simulink model "hovercraft_cascade_control"  (R2024a)
settings: Solver=VariableStepAuto  StartTime=0.0  StopTime=150  RelTol=1e-3
libraries: mpclib x1
settings Model: Creator=ettor  LastModifiedBy=ettor
settings SolverCC: MaxConsecutiveMinStep=100

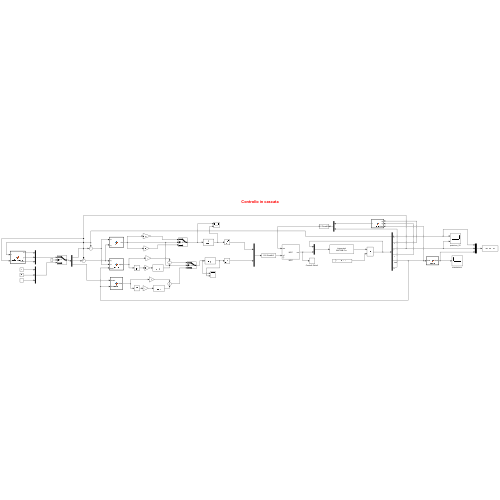
[thumbnail: Simulink's stored preview of the top-level diagram]
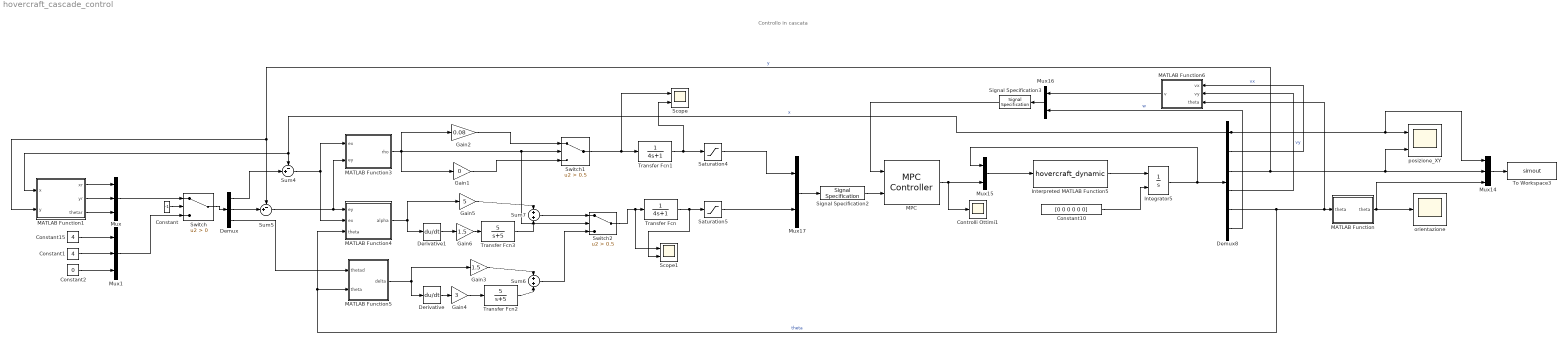
== system hovercraft_cascade_control ==
  note: Controllo in cascata
  Constant : Constant  Value=-1
  Constant1 : Constant  Value=4
  Constant10 : Constant  Value=[0 0 0 0 0 0]
  Constant15 : Constant  Value=4
  Constant2 : Constant  Value=0
  Controlli Ottimi1 : Scope
  Demux : Demux  Outputs=3
  Demux8 : Demux  Outputs=6
  Derivative : Derivative
  Derivative1 : Derivative
  Gain1 : Gain  Gain=0
  Gain2 : Gain  Gain=0.08
  Gain3 : Gain  Gain=1.5
  Gain4 : Gain  Gain=3
  Gain5 : Gain  Gain=5
  Gain6 : Gain  Gain=1.5
  Integrator5 : Integrator  InitialConditionSource=external
  Interpreted MATLAB Function5 : MATLABFcn  MATLABFcn=hovercraft_dynamic
  MATLAB Function : MATLAB Function  TreatAsAtomicUnit=on
  MATLAB Function1 : MATLAB Function  TreatAsAtomicUnit=on
  MATLAB Function3 : MATLAB Function  TreatAsAtomicUnit=on
  MATLAB Function4 : MATLAB Function  TreatAsAtomicUnit=on
  MATLAB Function5 : MATLAB Function  TreatAsAtomicUnit=on
  MATLAB Function6 : MATLAB Function  TreatAsAtomicUnit=on
  MPC : mpclib/MPC Controller  SCDEnableBlockLinearizationSpecification=on  mpcobj=mpc_simp  is_multiple=0  enable_value=0  return_u0=off  updateMPCinCallerWorkspace=on  md_inport=off  mv_inport=off  uref_inport=off  return_cost=off  return_mvseq=off  return_qpstatus=off  return_xseq=off  return_state=off  return_ovseq=off  state_inport=off  umin_inport=off  umax_inport=off  ymin_inport=off  ymax_inport=off  cc_inport=off  ywt_inport=off  uwt_inport=off  duwt_inport=off  rhoeps_inport=off  pm_inport=off  MaximumP=10  HorizonChoice=FixedHorizon  n_ts=0.05  n_p=80  n_mv=2  n_md=0  n_ud=0  n_mo=2  n_uo=0  BlockDataType=double  SampleTimeInherited=off  switch_inport=off
  Mux : Mux  Inputs=3
  Mux1 : Mux  Inputs=3
  Mux14 : Mux  Inputs=3
  Mux15 : Mux  Inputs=2
  Mux16 : Mux  Inputs=2
  Mux17 : Mux  Inputs=2
  Saturation4 : Saturate  UpperLimit=12  LowerLimit=-6
  Saturation5 : Saturate  UpperLimit=0.9  LowerLimit=-0.9
  Scope : Scope  NumInputPorts=2
  Scope1 : Scope  NumInputPorts=2
  Signal Specification2 : SignalSpecification  Dimensions=2
  Signal Specification3 : SignalSpecification  Dimensions=2
  Sum4 : Sum  Inputs=-+|
  Sum5 : Sum  Inputs=-+|
  Sum6 : Sum  Inputs=+|+
  Sum7 : Sum  Inputs=+|+
  Switch : Switch  Criteria=u2 > Threshold  SaturateOnIntegerOverflow=off  InputSameDT=off
  Switch1 : Switch  Criteria=u2 > Threshold  Threshold=0.5  SaturateOnIntegerOverflow=off  InputSameDT=off
  Switch2 : Switch  Criteria=u2 > Threshold  Threshold=0.5  SaturateOnIntegerOverflow=off  InputSameDT=off
  To Workspace3 : ToWorkspace  VariableName=simout  SaveFormat=Structure With Time  SampleTime=-1
      settings: Save2DSignal=2-D array (concatenate along first dimension)
  Transfer Fcn : TransferFcn  Denominator=[4 1]
  Transfer Fcn1 : TransferFcn  Denominator=[4 1]
  Transfer Fcn2 : TransferFcn  Numerator=5  Denominator=[1 5]
  Transfer Fcn3 : TransferFcn  Numerator=[5]  Denominator=[1 5]
  "orientazione " : Scope
  posizione_XY : Scope  NumInputPorts=2
  wires:
  Gain4/1 -> Transfer Fcn2/1
  Gain6/1 -> Transfer Fcn3/1
  Derivative1/1 -> Gain6/1
  Transfer Fcn2/1 -> Sum6/2
  Gain5/1 -> Sum7/1
  Demux8/5 -> MATLAB Function/1("theta "), MATLAB Function6/3(theta), MATLAB Function5/2(theta), MATLAB Function4/3(theta)  "theta"
  Mux15/1 -> Interpreted MATLAB Function5/1
  MPC/1 -> Controlli Ottimi1/1, Mux15/2
  Saturation5/1 -> Mux17/2
  Integrator5/1 -> Mux15/1, Demux8/1
  Demux8/6 -> Mux16/2  "w"
  Mux16/1 -> Signal Specification3/1
  Interpreted MATLAB Function5/1 -> Integrator5/1
  Saturation4/1 -> Mux17/1
  Transfer Fcn/1 -> Scope1/2, Saturation5/1
  Constant10/1 -> Integrator5/2
  Demux8/4 -> MATLAB Function6/2(vy)  "vy"
  Mux14/1 -> To Workspace3/1
  Demux8/3 -> posizione_XY/2, Mux14/2, Sum5/1, MATLAB Function1/2(y)  "y"
  Demux8/2 -> MATLAB Function6/1(vx)  "vx"
  MATLAB Function5/1(delta) -> Gain3/1, Derivative/1
  Mux17/1 -> Signal Specification2/1
  Gain3/1 -> Sum6/1
  Transfer Fcn1/1 -> Scope/2, Saturation4/1
  Demux8/1 -> Mux14/1, posizione_XY/1, MATLAB Function1/1(x), Sum4/1  "x"
  Transfer Fcn3/1 -> Sum7/2
  Signal Specification2/1 -> MPC/2
  Derivative/1 -> Gain4/1
  Switch2/1 -> Scope1/1, Transfer Fcn/1
  Sum7/1 -> Switch2/1
  MATLAB Function3/1(rho) -> Gain2/1, Switch2/2, Switch1/2, Gain1/1
  MATLAB Function4/1(alpha) -> Gain5/1, Derivative1/1
  Gain2/1 -> Switch1/1
  Switch1/1 -> Scope/1, Transfer Fcn1/1
  Sum6/1 -> Switch2/3
  Gain1/1 -> Switch1/3
  Sum4/1 -> MATLAB Function4/2(ex), MATLAB Function3/1(ex)
  Sum5/1 -> MATLAB Function4/1(ey), MATLAB Function3/2(ey)
  Demux/2 -> Sum5/2
  Demux/1 -> Sum4/2
  MATLAB Function1/1(xr) -> Mux/1
  MATLAB Function1/2(yr) -> Mux/2
  MATLAB Function1/3(thetar) -> Mux/3
  Mux/1 -> Switch/1
  Constant1/1 -> Mux1/2
  Constant15/1 -> Mux1/1
  Constant2/1 -> Mux1/3
  Mux1/1 -> Switch/3
  Constant/1 -> Switch/2
  Switch/1 -> Demux/1
  Demux/3 -> MATLAB Function5/1(thetad)
  MATLAB Function/1(theta) -> "orientazione "/1, Mux14/3
  MATLAB Function6/1(v) -> Mux16/1
  Signal Specification3/1 -> MPC/1

== matlab function hovercraft_cascade_control/MATLAB Function1 ==
  data: x input; xr output; y input; yr output; thetar output
function [xr, yr, thetar] = path_tracking(x, y)
    
    % Variabili Globali 
    persistent x_path y_path N lookahead

    %Definizione percorso  
    if isempty(x_path)
        %discretizzazione percorso 
        R = 2; xc = 2; yc = 2;
        theta = linspace(0, 2*pi, 1000);
        x_path = xc + R*cos(theta);
        y_path = yc + R*sin(theta);
        N = length(x_path);

        % Lookahead in metri → convertito in n° punti
        lookahead_distance = 1;  
        point_spacing = (2*pi*R) / N;
        lookahead = floor(lookahead_distance / point_spacing);
    end

    % Trova punto più vicino
    distances = (x_path - x).^2 + (y_path - y).^2;
    [~, idx] = min(distances);

    % Punto lookahead
    idx_look = mod(idx + lookahead - 1, N) + 1; %mod per indice circolare, mod(1001,1000)=1;  (Matlab parte da 1 non da 0) 
    xr = x_path(idx_look);
    yr = y_path(idx_look);

    % Orientamento tangente
    idx_next = mod(idx_look + 1 - 1, N) + 1;
    dx = x_path(idx_next) - x_path(idx_look);
    dy = y_path(idx_next) - y_path(idx_look);
    thetar = atan2(dy, dx);

end

== matlab function hovercraft_cascade_control/MATLAB Function ==
  data: theta input; theta output
function theta = norm(theta)
    theta=atan2(sin(theta),cos(theta)); 
end

== matlab function hovercraft_cascade_control/MATLAB Function3 ==
  data: ex input; rho output; ey input
function rho = rho(ex,ey)
    rho=sqrt(ex^2+ey^2); 
end

== matlab function hovercraft_cascade_control/MATLAB Function4 ==
  data: ey input; ex input; alpha output; theta input
function alpha = alpha(ey,ex,theta)
    alpha = atan2(ey, ex) - theta;
    alpha = atan2(sin(alpha), cos(alpha));
end

== matlab function hovercraft_cascade_control/MATLAB Function5 ==
  data: thetad input; delta output; theta input
function delta = delta(thetad, theta)
    
    
    delta = thetad - theta;

    

    
    delta= atan2(sin(delta), cos(delta));
    
end

== matlab function hovercraft_cascade_control/MATLAB Function6 ==
  data: vx input; v output; vy input; theta input
function v = fcn(vx, vy, theta)
    v = vx*cos(theta) + vy*sin(theta); 
    
end
